simulink model "dsp_event_test"  (R2021b)
settings: Solver=ode45  StartTime=0.0  StopTime=80e-6  MaxStep=7.3e-6  RelTol=1e-7  AbsTol=1e-9
values from neighbouring files (symbols this model uses):
  config = [10 1514 1000]    [validate_m1.m]
  event_file = fullfile(folder,[name '_events.csv'])    [event_case.m]    (also in pfc_case.m)
settings Model: Creator=yangs  LastModifiedBy=yangs
settings SolverCC: ZeroCrossControl=EnableAll  ZeroCrossAlgorithm=Adaptive

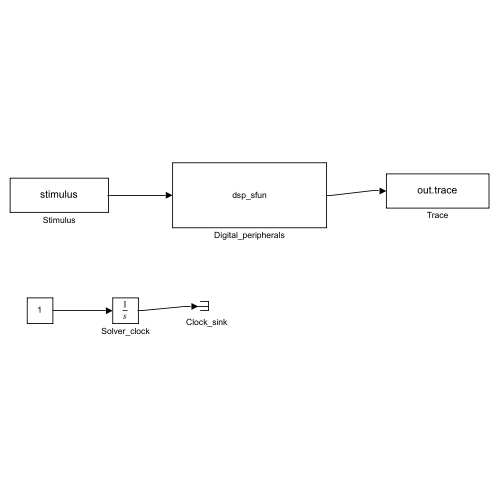
[thumbnail: Simulink's stored preview of the top-level diagram]
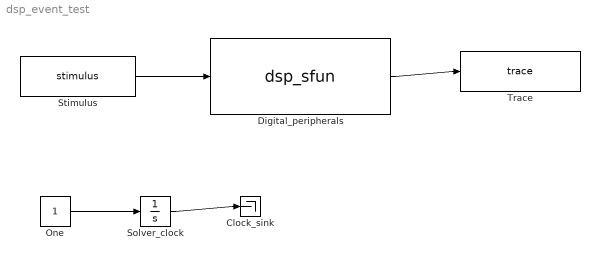
== system dsp_event_test ==
  Clock_sink : Terminator
  Digital_peripherals : S-Function  FunctionName=dsp_sfun  Parameters=config,event_file  SFunctionDeploymentMode=off  EnableBusSupport=off
  One : Constant
  Solver_clock : Integrator
  Stimulus : FromWorkspace  VariableName=stimulus  Interpolate=off  OutputAfterFinalValue=Holding final value
  Trace : ToWorkspace  VariableName=trace  SaveFormat=Structure With Time  SampleTime=-1
  wires:
  Stimulus/1 -> Digital_peripherals/1
  Digital_peripherals/1 -> Trace/1
  One/1 -> Solver_clock/1
  Solver_clock/1 -> Clock_sink/1
